simulink model "tp"  (R2025b)
settings: Solver=VariableStepAuto  StartTime=0.0  StopTime=10.0  FixedStep=0.0001  MaxStep=0.001  RelTol=1e-4
undefined symbols (not defined in the file): A, a1, a2, a3, a4, b, C, C_add, gamma, K
settings Model: Creator=Nickolay  LastModifiedBy=Nickolay

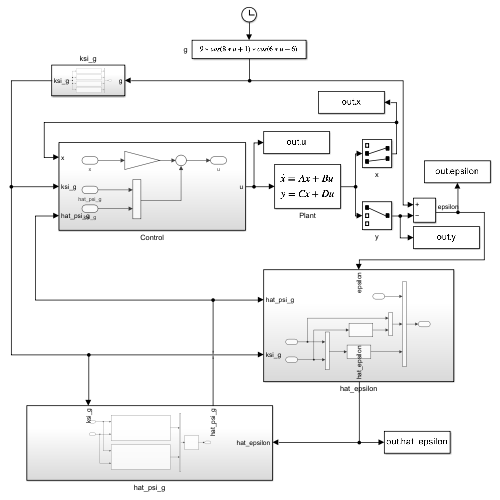
[thumbnail: Simulink's stored preview of the top-level diagram]
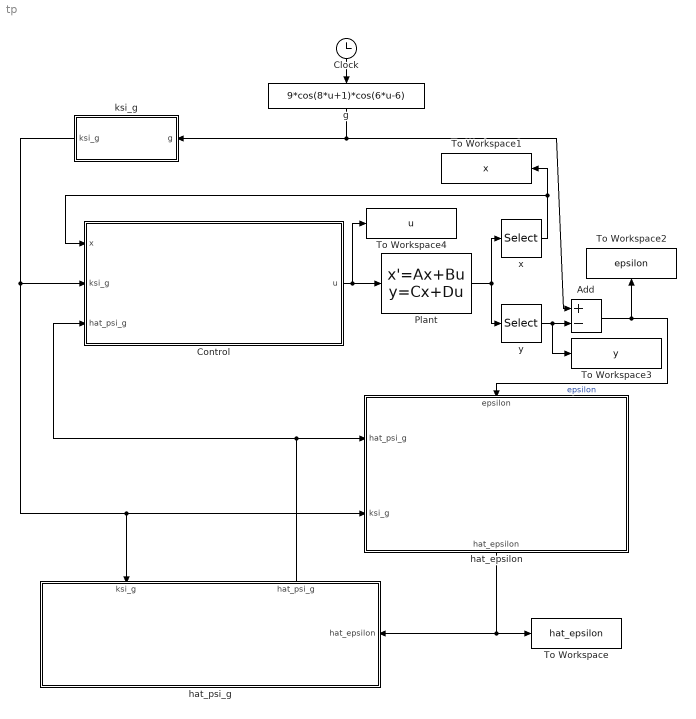
== system tp ==
  Add : Sum  Inputs=+-
  Clock : Clock
  Control : Subsystem
  Plant : StateSpace  A=A  B=b  C=C_add  D=zeros(3,1)  InitialCondition=[0 0]
  To Workspace : ToWorkspace  VariableName=hat_epsilon  SaveFormat=Timeseries  SampleTime=-1
  To Workspace1 : ToWorkspace  VariableName=x  SaveFormat=Timeseries  SampleTime=-1
  To Workspace2 : ToWorkspace  VariableName=epsilon  SaveFormat=Timeseries  SampleTime=-1
  To Workspace3 : ToWorkspace  VariableName=y  SaveFormat=Timeseries  SampleTime=-1
  To Workspace4 : ToWorkspace  VariableName=u  SaveFormat=Timeseries  SampleTime=-1
  g : Fcn  Expr=9*cos(8*u+1)*cos(6*u-6)
  hat_epsilon : Subsystem
      settings: PortSchema="{\"entries\":[{\"content\":{\"sides\":[{\"content\":{\"connectorIds\":[\"In1\",\"In2\"]},\"type\":\"ConnectorPlacement.EquallySpacedRectSide\",\"uuid\":\"48c1e5cb-92d9-4787-8f42-40c39f9dea44\"},{\"content\":{\"side\":\"RIGHT\"},\"type\":\"ConnectorPlacement.EquallySpacedRectSide\",\"uuid\":\"80026722-3371-4a94-89dc-394597967272\"},{\"content\":{\"connectorIds\":[\"In3\"],\"side\":\"TOP\"},\"type\":\"ConnectorPlacement.EquallySpacedRectSide\",\"uuid\":\"1bbb4d7a-7147-4365-9996-4f5c12e2a758\"},{\"content\":{\"connectorIds\":[\"Out1\"],\"side\":\"BOTTOM\"},\"type\":\"ConnectorPlacement.EquallySpacedRectSide\",\"uuid\":\"4436094d-444e-4d5f-bb69-fcc560e0543c\"}]},\"type\":\"ConnectorPlacement.EquallySpacedConnector\",\"uuid\":\"78f5ac4d-70a5-40fc-842a-17a7a2e66dbb\"}],\"packageUris\":[\"http://schema.mathworks.com/mf0/Connector/R2020b\"],\"version\":\"1.0\"}"
  hat_psi_g : Subsystem
      settings: PortSchema="{\"entries\":[{\"content\":{\"sides\":[{\"content\":{},\"type\":\"ConnectorPlacement.EquallySpacedRectSide\",\"uuid\":\"8c541289-e3ac-4623-ad1a-56e6ff51ab1e\"},{\"content\":{\"connectorIds\":[\"In2\"],\"side\":\"RIGHT\"},\"type\":\"ConnectorPlacement.EquallySpacedRectSide\",\"uuid\":\"641fd83c-68a9-4881-af8c-11f9afc4a7f8\"},{\"content\":{\"connectorIds\":[\"In1\",\"Out1\"],\"side\":\"TOP\"},\"type\":\"ConnectorPlacement.EquallySpacedRectSide\",\"uuid\":\"95517ae1-b1b5-4683-be3c-670cc6992aa1\"},{\"content\":{\"side\":\"BOTTOM\"},\"type\":\"ConnectorPlacement.EquallySpacedRectSide\",\"uuid\":\"61675a38-f01b-426f-af21-1a3bcddbeb78\"}]},\"type\":\"ConnectorPlacement.EquallySpacedConnector\",\"uuid\":\"f599e1e7-6248-41df-84f3-802213366fe6\"}],\"packageUris\":[\"http://schema.mathworks.com/mf0/Connector/R2020b\"],\"version\":\"1.0\"}"
  ksi_g : Subsystem
  x : Selector  InputPortWidth=3  IndexOptions=Index vector (dialog)  Indices=[2 3]  OutputSizes=1
  y : Selector  InputPortWidth=3  IndexOptions=Index vector (dialog)  Indices=1  OutputSizes=1
  wires:
  Control/1(u) -> To Workspace4/1, Plant/1
  Plant/1 -> x/1, y/1
  x/1 -> To Workspace1/1, Control/1(x)
  g/1 -> Add/1, ksi_g/1(g)
  Add/1 -> hat_epsilon/3(epsilon), To Workspace2/1  "epsilon"
  ksi_g/1(ksi_g) -> hat_epsilon/2(ksi_g), hat_psi_g/1(ksi_g), Control/2(ksi_g)
  Clock/1 -> g/1
  hat_epsilon/1(hat_epsilon) -> To Workspace/1, hat_psi_g/2(hat_epsilon)
  hat_psi_g/1(hat_psi_g) -> Control/3(hat_psi_g), hat_epsilon/1(hat_psi_g)
  y/1 -> To Workspace3/1, Add/2

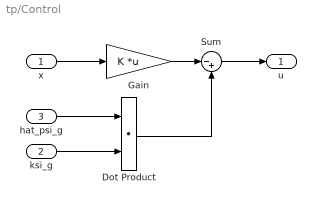
== system tp/Control ==
  x : Inport
  ksi_g : Inport  Port=2
  hat_psi_g : Inport  Port=3
  Dot Product : DotProduct  OutDataTypeStr=Inherit: Inherit via internal rule
  Gain : Gain  Gain=K  Multiplication=Matrix(K*u) (u vector)
  Sum : Sum  Inputs=|-+
  u : Outport
  wires:
  x/1 -> Gain/1
  Gain/1 -> Sum/1
  Sum/1 -> u/1
  hat_psi_g/1 -> Dot Product/1
  ksi_g/1 -> Dot Product/2
  Dot Product/1 -> Sum/2

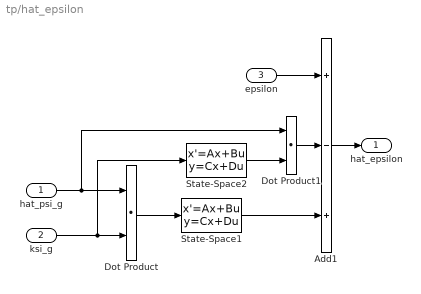
== system tp/hat_epsilon ==
  hat_psi_g : Inport
  ksi_g : Inport  Port=2
  epsilon : Inport  Port=3
  Add1 : Sum  Inputs=+-+
  Dot Product : DotProduct  OutDataTypeStr=Inherit: Inherit via internal rule
  Dot Product1 : DotProduct  OutDataTypeStr=Inherit: Inherit via internal rule
  State-Space1 : StateSpace  A=A-b*K  B=b  C=C  D=0  InitialCondition=zeros(2,1)
  State-Space2 : StateSpace  A=kron(eye(4), A-b*K)  B=kron(eye(4), b)  C=kron(eye(4), C)  D=zeros(4,4)  InitialCondition=zeros(8,1)
  hat_epsilon : Outport
  wires:
  epsilon/1 -> Add1/1
  Dot Product/1 -> State-Space1/1
  hat_psi_g/1 -> Dot Product1/1, Dot Product/1
  State-Space1/1 -> Add1/3
  ksi_g/1 -> State-Space2/1, Dot Product/2
  State-Space2/1 -> Dot Product1/2
  Dot Product1/1 -> Add1/2
  Add1/1 -> hat_epsilon/1

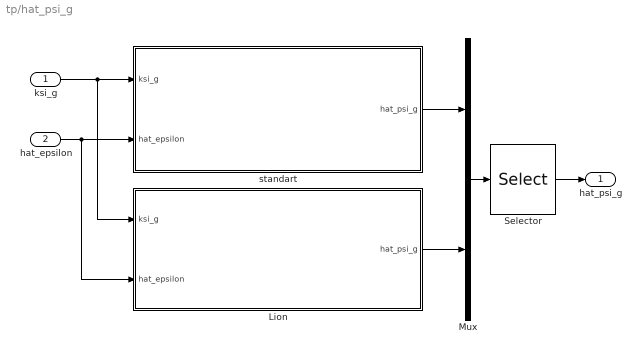
== system tp/hat_psi_g ==
  ksi_g : Inport
  hat_epsilon : Inport  Port=2
  Lion : Subsystem
  Mux : Mux  Inputs=2
  Selector : Selector  InputPortWidth=8  IndexOptions=Index vector (dialog)  Indices=[1 2 3 4]  OutputSizes=1
  standart : Subsystem
  hat_psi_g : Outport
  wires:
  Selector/1 -> hat_psi_g/1
  ksi_g/1 -> Lion/1(ksi_g), standart/1(ksi_g)
  Mux/1 -> Selector/1
  standart/1(hat_psi_g) -> Mux/1
  hat_epsilon/1 -> Lion/2(hat_epsilon), standart/2(hat_epsilon)
  Lion/1(hat_psi_g) -> Mux/2

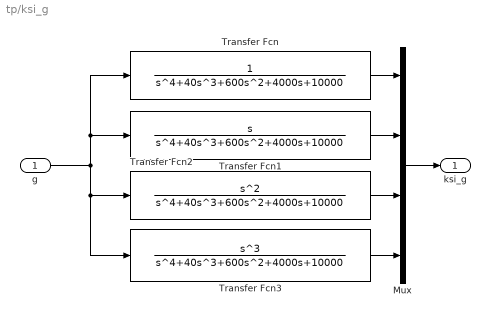
== system tp/ksi_g ==
  g : Inport
  Mux : Mux
  Transfer Fcn : TransferFcn  Denominator=[1 40 600 4000 10000]
  Transfer Fcn1 : TransferFcn  Numerator=[1 0]  Denominator=[1 40 600 4000 10000]
  Transfer Fcn2 : TransferFcn  Numerator=[1 0 0]  Denominator=[1 40 600 4000 10000]
  Transfer Fcn3 : TransferFcn  Numerator=[1 0 0 0]  Denominator=[1 40 600 4000 10000]
  ksi_g : Outport
  wires:
  g/1 -> Transfer Fcn/1, Transfer Fcn1/1, Transfer Fcn3/1, Transfer Fcn2/1
  Transfer Fcn/1 -> Mux/1
  Transfer Fcn1/1 -> Mux/2
  Transfer Fcn2/1 -> Mux/3
  Transfer Fcn3/1 -> Mux/4
  Mux/1 -> ksi_g/1

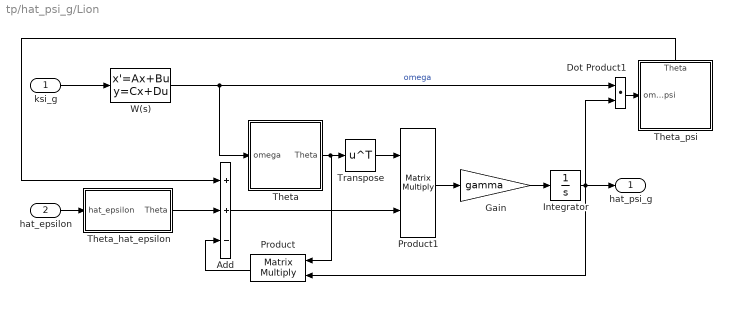
== system tp/hat_psi_g/Lion ==
  ksi_g : Inport
  hat_epsilon : Inport  Port=2
  Add : Sum  Inputs=++-
  Dot Product1 : DotProduct  OutDataTypeStr=Inherit: Inherit via internal rule
  Gain : Gain  Gain=gamma
  Integrator : Integrator
  Product : Product  Multiplication=Matrix(*)
  Product1 : Product  Multiplication=Matrix(*)
  Theta : Subsystem
  Theta_hat_epsilon : Subsystem
  Theta_psi : Subsystem
      settings: PortSchema="{\"entries\":[{\"content\":{\"sides\":[{\"content\":{\"connectorIds\":[\"In1\"]},\"type\":\"ConnectorPlacement.EquallySpacedRectSide\",\"uuid\":\"8849c319-b507-4d19-bda6-458101ea9b3a\"},{\"content\":{\"side\":\"RIGHT\"},\"type\":\"ConnectorPlacement.EquallySpacedRectSide\",\"uuid\":\"21821828-ec8e-4949-8613-8277e754c5a8\"},{\"content\":{\"connectorIds\":[\"Out1\"],\"side\":\"TOP\"},\"type\":\"ConnectorPlacement.EquallySpacedRectSide\",\"uuid\":\"c135362d-0868-465b-82eb-a2e45883022f\"}]},\"type\":\"ConnectorPlacement.EquallySpacedConnector\",\"uuid\":\"cefe3068-61de-45df-911b-88d28fa18064\"}],\"packageUris\":[\"http://schema.mathworks.com/mf0/Connector/R2020b\"],\"version\":\"1.0\"}"
  Transpose : Math  Operator=transpose
  W(s) : StateSpace  A=kron(eye(4), A-b*K)  B=kron(eye(4), b)  C=kron(eye(4), C)  D=zeros(4,4)  InitialCondition=zeros(8,1)
  hat_psi_g : Outport
  wires:
  ksi_g/1 -> W(s)/1
  W(s)/1 -> Theta/1(omega), Dot Product1/1  "omega"
  Theta/1(Theta) -> Product/1, Transpose/1
  Product1/1 -> Gain/1
  Add/1 -> Product1/2
  hat_epsilon/1 -> Theta_hat_epsilon/1(hat_epsilon)
  Dot Product1/1 -> Theta_psi/1(omega_psi)
  Theta_psi/1(Theta) -> Add/1
  Theta_hat_epsilon/1(Theta) -> Add/2
  Gain/1 -> Integrator/1
  Integrator/1 -> Product/2, hat_psi_g/1, Dot Product1/2
  Product/1 -> Add/3
  Transpose/1 -> Product1/1

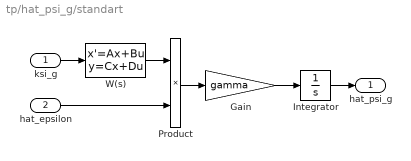
== system tp/hat_psi_g/standart ==
  ksi_g : Inport
  hat_epsilon : Inport  Port=2
  Gain : Gain  Gain=gamma
  Integrator : Integrator  InitialCondition=zeros(4,1)
  Product : Product
  W(s) : StateSpace  A=kron(eye(4), A-b*K)  B=kron(eye(4), b)  C=kron(eye(4), C)  D=zeros(4,4)  InitialCondition=zeros(8,1)
  hat_psi_g : Outport
  wires:
  ksi_g/1 -> W(s)/1
  Integrator/1 -> hat_psi_g/1
  Product/1 -> Gain/1
  Gain/1 -> Integrator/1
  W(s)/1 -> Product/1
  hat_epsilon/1 -> Product/2

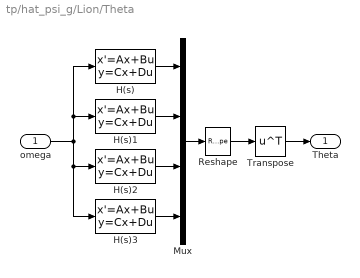
== system tp/hat_psi_g/Lion/Theta ==
  omega : Inport
  H(s) : StateSpace  A=-a1*eye(4)  B=a1*eye(4)  C=eye(4)  D=zeros(4,4)  InitialCondition=0
  H(s)1 : StateSpace  A=-a2*eye(4)  B=a2*eye(4)  C=eye(4)  D=zeros(4,4)  InitialCondition=0
  H(s)2 : StateSpace  A=-a3*eye(4)  B=a3*eye(4)  C=eye(4)  D=zeros(4,4)  InitialCondition=0
  H(s)3 : StateSpace  A=-a4*eye(4)  B=a4*eye(4)  C=eye(4)  D=zeros(4,4)  InitialCondition=0
  Mux : Mux
  Reshape : Reshape  OutputDimensionality=Customize  OutputDimensions=[4,4]
  Transpose : Math  Operator=transpose
  Theta : Outport
  wires:
  H(s)/1 -> Mux/1
  H(s)2/1 -> Mux/3
  H(s)3/1 -> Mux/4
  H(s)1/1 -> Mux/2
  omega/1 -> H(s)3/1, H(s)2/1, H(s)/1, H(s)1/1
  Reshape/1 -> Transpose/1
  Transpose/1 -> Theta/1
  Mux/1 -> Reshape/1

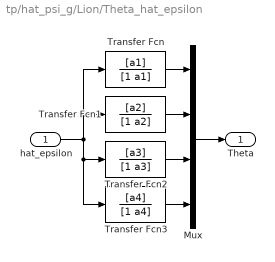
== system tp/hat_psi_g/Lion/Theta_hat_epsilon ==
  hat_epsilon : Inport
  Mux : Mux
  Transfer Fcn : TransferFcn  Numerator=[a1]  Denominator=[1 a1]
  Transfer Fcn1 : TransferFcn  Numerator=[a2]  Denominator=[1 a2]
  Transfer Fcn2 : TransferFcn  Numerator=[a3]  Denominator=[1 a3]
  Transfer Fcn3 : TransferFcn  Numerator=[a4]  Denominator=[1 a4]
  Theta : Outport
  wires:
  Transfer Fcn/1 -> Mux/1
  Transfer Fcn2/1 -> Mux/3
  Transfer Fcn3/1 -> Mux/4
  Transfer Fcn1/1 -> Mux/2
  hat_epsilon/1 -> Transfer Fcn3/1, Transfer Fcn2/1, Transfer Fcn1/1, Transfer Fcn/1
  Mux/1 -> Theta/1

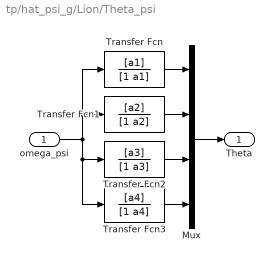
== system tp/hat_psi_g/Lion/Theta_psi ==
  omega_psi : Inport
  Mux : Mux
  Transfer Fcn : TransferFcn  Numerator=[a1]  Denominator=[1 a1]
  Transfer Fcn1 : TransferFcn  Numerator=[a2]  Denominator=[1 a2]
  Transfer Fcn2 : TransferFcn  Numerator=[a3]  Denominator=[1 a3]
  Transfer Fcn3 : TransferFcn  Numerator=[a4]  Denominator=[1 a4]
  Theta : Outport
  wires:
  Transfer Fcn/1 -> Mux/1
  Transfer Fcn2/1 -> Mux/3
  Transfer Fcn3/1 -> Mux/4
  Transfer Fcn1/1 -> Mux/2
  omega_psi/1 -> Transfer Fcn3/1, Transfer Fcn2/1, Transfer Fcn1/1, Transfer Fcn/1
  Mux/1 -> Theta/1
